simulink model "fft_biplex_real_2x_test"  (Simulink 7.4)
settings: Solver=VariableStepDiscrete  StartTime=0.0  StopTime=256  RelTol=1e-3
libraries: xbsIndex_r4 x519, casper_library_misc x26, casper_library_delays x7, casper_library_ffts_twiddle x1, simulink x1
(part 6 of 6)

== system fft_biplex_real_2x_test/fft_biplex_real_2x/biplex_core/fft_stage_5/butterfly_direct/twiddle_general_3mult/coeff_gen ==
  rst : Inport
  Counter : xbsIndex_r4/Counter  cnt_type=Free Running  cnt_to=Inf  operation=Up  start_count=0  cnt_by_val=1  arith_type=Unsigned  n_bits=4  bin_pt=0  load_pin=off  rst=on  en=off  explicit_period=on  period=1  dbl_ovrd=off  use_behavioral_HDL=off  implementation=Fabric  block_type=counter
      settings: block_version=11.4
  ROM : xbsIndex_r4/ROM  depth=16  initVector="[1                                      0                       0.70709228515625                      -0.70709228515625                       0.92388916015625                       -0.3826904296875                        0.3826904296875                      -0.92388916015625                       0.98077392578125                     -0.195098876953125                      0.555572509765625                      -0.83148193359375                       0.83148193359375                     -0.555572509765625                      0.195098876953125                      -0.98077392578125]"  distributed_mem=Block RAM  rst=off  init_reg=0  en=off  latency=2  arith_type="Signed  (2's comp)"  n_bits=17  bin_pt=15  dbl_ovrd=off  optimize=Area  use_rpm=on  block_type=sprom
      settings: block_version=11.4
  ROM1 : xbsIndex_r4/ROM  depth=16  initVector="[0                                     -1                      -0.70709228515625                      -0.70709228515625                       -0.3826904296875                      -0.92388916015625                      -0.92388916015625                       -0.3826904296875                     -0.195098876953125                      -0.98077392578125                      -0.83148193359375                     -0.555572509765625                     -0.555572509765625                      -0.83148193359375                      -0.98077392578125                     -0.195098876953125]"  distributed_mem=Block RAM  rst=off  init_reg=0  en=off  latency=2  arith_type="Signed  (2's comp)"  n_bits=17  bin_pt=15  dbl_ovrd=off  optimize=Area  use_rpm=on  block_type=sprom
      settings: block_version=11.4
  Slice : xbsIndex_r4/Slice  nbits=4  boolean_output=off  mode=Upper Bit Location + Width  bit1=0  base1=MSB of Input  bit0=0  base0=LSB of Input  dbl_ovrd=off  block_type=slice
  ri_to_c : casper_library_misc/ri_to_c  SystemSampleTime=-1
  w : Outport
  wires:
  ri_to_c/1 -> w/1
  rst/1 -> Counter/1
  Counter/1 -> Slice/1
  Slice/1 -> ROM/1, ROM1/1
  ROM/1 -> ri_to_c/1
  ROM1/1 -> ri_to_c/2
